simulink model "HPPC"  (R2026a)
settings: Solver=FixedStepDiscrete  StopTime=inf  FixedStep=Ts
model workspace (MATLAB code in the model file):
  | % Defaults for standalone use and code generation, from HPP_parameters.
  | % In HPP.slx the Model block passes p.ctrl.hppc.par as the argument "par".
  | pDefault = HPP_parameters();
  | Ts  = pDefault.ctrl.hppc.Ts;    % [s] fixed sample time
  | par = pDefault.ctrl.hppc.par;   % tunable parameters (model argument)
  | clear pDefault
libraries: simulink x5, slpidlib x2, sl_discontinuities x1
Description:
  | HPP controller (stage 5, Energinet DK1): P set-point with ramp rate constraint, frequency response (LFSM-O, LFSM-U, optional FSM with reserve; Frqflag) added after the ramp limit, export limit; closed-loop P at the POC (PI on P_target - P_poc, target fed forward, Pflag); SOC-aware BESS limits; dispatch: wind and PV at available power, the BESS balances, wind and PV curtailed when the BESS cannot absorb more. Q control (Q_ref), voltage control (Vref, slope Vslope) or power factor control (PF) at the POC with PI (Qflag, RefFlag 0 / 1 / 2), Q order split over the plants by rating. Both PIs frozen in a voltage dip. Per unit on p.ctrl.hppc.Pbase. Parameters: model argument par (= p.ctrl.hppc.par, from p.hppc).
settings Model: ParameterArgumentNames=par  Creator=kjaer  LastModifiedBy=kjaer

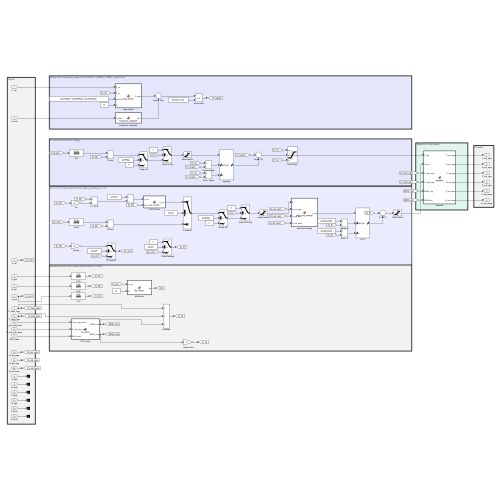
[thumbnail: Simulink's stored preview of the top-level diagram]
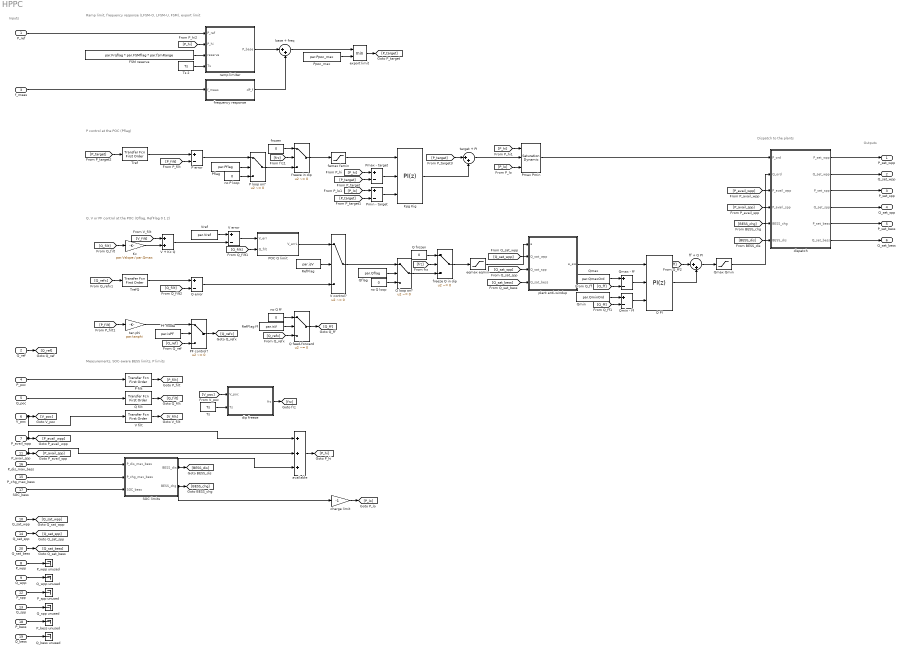
== system HPPC ==
  note: Inputs
  note: Ramp limit, frequency response (LFSM-O, LFSM-U, FSM), export limit
  note: P control at the POC (Pflag)
  note: Q, V or PF control at the POC (Qflag, RefFlag 0 1 2)
  note: Measurements, SOC-aware BESS limits, P limits
  note: Dispatch to the plants
  note: Outputs
  P_ref : Inport  OutDataTypeStr=double  PortDimensions=1  SampleTime=Ts
  Q_ref : Inport  Port=2  OutDataTypeStr=double  PortDimensions=1  SampleTime=Ts
  f_meas : Inport  Port=3  OutDataTypeStr=double  PortDimensions=1  SampleTime=Ts
  P_poc : Inport  Port=4  OutDataTypeStr=double  PortDimensions=1  SampleTime=Ts
  Q_poc : Inport  Port=5  OutDataTypeStr=double  PortDimensions=1  SampleTime=Ts
  V_poc : Inport  Port=6  OutDataTypeStr=double  PortDimensions=1  SampleTime=Ts
  P_avail_wpp : Inport  Port=7  OutDataTypeStr=double  PortDimensions=1  SampleTime=Ts
  P_wpp : Inport  Port=8  OutDataTypeStr=double  PortDimensions=1  SampleTime=Ts
  Q_wpp : Inport  Port=9  OutDataTypeStr=double  PortDimensions=1  SampleTime=Ts
  Q_sat_wpp : Inport  Port=10  OutDataTypeStr=double  PortDimensions=1  SampleTime=Ts
  P_avail_spp : Inport  Port=11  OutDataTypeStr=double  PortDimensions=1  SampleTime=Ts
  P_spp : Inport  Port=12  OutDataTypeStr=double  PortDimensions=1  SampleTime=Ts
  Q_spp : Inport  Port=13  OutDataTypeStr=double  PortDimensions=1  SampleTime=Ts
  Q_sat_spp : Inport  Port=14  OutDataTypeStr=double  PortDimensions=1  SampleTime=Ts
  P_chg_max_bess : Inport  Port=15  OutDataTypeStr=double  PortDimensions=1  SampleTime=Ts
  P_dis_max_bess : Inport  Port=16  OutDataTypeStr=double  PortDimensions=1  SampleTime=Ts
  SOC_bess : Inport  Port=17  OutDataTypeStr=double  PortDimensions=1  SampleTime=Ts
  P_bess : Inport  Port=18  OutDataTypeStr=double  PortDimensions=1  SampleTime=Ts
  Q_bess : Inport  Port=19  OutDataTypeStr=double  PortDimensions=1  SampleTime=Ts
  Q_sat_bess : Inport  Port=20  OutDataTypeStr=double  PortDimensions=1  SampleTime=Ts
  FSM reserve : Constant  Value=par.Frqflag * par.FSMflag * par.fsmRange
  Kc : Gain  Gain=par.Vslope / par.Qmax
  Kpg Kig : slpidlib/PID Controller  Controller=PI  Form=Parallel  TimeDomain=Discrete-time  UseExternalTs=off  SampleTime=-1  IntegratorMethod=Forward Euler  FilterMethod=Forward Euler  ControllerParametersSource=internal  P=par.Kpg  I=par.Kig  UseKiTs=off  D=0  UseExternalDerivativeSource=off  N=100  UseFilter=on  TunerSelectOption=Transfer Function Based (PID Tuner App)  InitialConditionSource=internal  InitialConditionForIntegrator=0  InitialConditionForFilter=0  DifferentiatorICPrevScaledInput=0  ExternalReset=none  TrackingMode=off  Kt=1  LimitOutput=on  SatLimitsSource=external  UpperSaturationLimit=inf  LowerSaturationLimit=-inf  LinearizeAsGain=off  AntiWindupMode=clamping  Kb=1  LimitIntegrator=off  UpperIntegratorSaturationLimit=inf  LowerIntegratorSaturationLimit=-inf  POutMin=[]  POutMax=[]  IOutMin=[]  IOutMax=[]  DOutMin=[]  DOutMax=[]  NOutMin=[]  NOutMax=[]  SumOutMin=[]  SumOutMax=[]  SaturationOutMin=[]  SaturationOutMax=[]  PParamMin=[]  PParamMax=[]  IParamMin=[]  IParamMax=[]  DParamMin=[]  DParamMax=[]  NParamMin=[]  NParamMax=[]  KbParamMin=[]  KbParamMax=[]  KtParamMin=[]  KtParamMax=[]  KbOutMin=[]  KbOutMax=[]  KtOutMin=[]  KtOutMax=[]  IntegratorOutMin=[]  IntegratorOutMax=[]  FilterOutMin=[]  FilterOutMax=[]  SumI1OutMin=[]  SumI1OutMax=[]  SumI2OutMin=[]  SumI2OutMax=[]  SumI3OutMin=[]  SumI3OutMax=[]  SumI4OutMin=[]  SumI4OutMax=[]  SumDOutMin=[]  SumDOutMax=[]  DifferentiatorOutMin=[]  DifferentiatorOutMax=[]  FilterDiffOutCoefMin=[]  FilterDiffOutCoefMax=[]  ReciprocalOutMin=[]  ReciprocalOutMax=[]  SumDenOutMin=[]  SumDenOutMax=[]  SumNumOutMin=[]  SumNumOutMax=[]  DivideOutMin=[]  DivideOutMax=[]  UdiffTsProdOutMin=[]  UdiffTsProdOutMax=[]  NTsProdOutMin=[]  NTsProdOutMax=[]  UintegralTsProdOutMin=[]  UintegralTsProdOutMax=[]  UngainTsProdOutMin=[]  UngainTsProdOutMax=[]  ClampingZeroOutDataTypeStr=Inherit: Inherit via back propagation  ClampingZeroOutMin=[]  ClampingZeroOutMax=[]  FilterDenConstantOutDataTypeStr=Inherit: Inherit via back propagation  FilterDenConstantOutMin=[]  FilterDenConstantOutMax=[]  PCopyOutDataTypeStr=Inherit: Inherit via back propagation  PCopyOutMin=[]  PCopyOutMax=[]  NCopyOutDataTypeStr=Inherit: Inherit via back propagation  NCopyOutMin=[]  NCopyOutMax=[]  IntegratorContinuousStateAttributes=''  IntegratorStateMustResolveToSignalObject=off  IntegratorRTWStateStorageClass=Auto  FilterContinuousStateAttributes=''  FilterStateMustResolveToSignalObject=off  FilterRTWStateStorageClass=Auto  ParallelPVariant=InternalParameters  IdealPVariant=Disabled  IVariant=InternalParameters  DVariant=Disabled  IntegratorVariant=Discrete  SatVariant=External  AWVariant=DiscClampingParallel  PCopyVariant=Disabled  TRVariant=Disabled  FdbkBlocksVariant=Forward  IdealPFdbkVariant=Disabled  SatFdbkVariant=Disabled  DerivativeFilterVariant=Disabled  NVariant=Disabled  NCopyVariant=Disabled_SignalSpec  FilterICVariant=Disabled  IntegratorICVariant=InternalICs  ExternalResetVariant=Disabled  TRSumVariant=Passthrough  SumFdbkVariant=Disabled  SumVariant=Sum_PI  TsampFilterVariant=InternalTs  TsampNgainVariant=Passthrough  TsampIntegralVariant=Disabled_SignalSpec  ExternalSaturationOutDataTypeStr=Inherit: Same as second input  DerivativeSourceVariant=Disabled  PreIntVariant=InternalPreInt
      settings: LibrarySourceBlock=simulink/Discrete/Discrete PID Controller
  P error : Sum  Inputs=+-
  P filt : simulink/Discrete/Transfer Fcn First Order  PoleZ=1 - Ts/par.Tp  ICPrevOutput=0  DoSatur=off
  P loop on? : Switch  Criteria=u2 ~= 0  SaturateOnIntegerOverflow=off  InputSameDT=off
  PF control? : Switch  Criteria=u2 ~= 0  SaturateOnIntegerOverflow=off  InputSameDT=off
  PF mode : Constant  Value=par.isPF
  POC Q limit : MATLAB Function  TreatAsAtomicUnit=on
  P_bess unused : Terminator
  P_spp unused : Terminator
  P_wpp unused : Terminator
  Pflag : Constant  Value=par.Pflag
  Pmax - target : Sum  Inputs=+-
  Pmax Pmin : sl_discontinuities/Saturation Dynamic  OutMin=[]  OutMax=[]  OutDataTypeStr=Inherit: Same as second input  OutDataType=fixdt(1, 16)  OutScaling=2^-10  DoSatur=off
      settings: LibrarySourceBlock=|
      | simulink/Discontinuities/Saturation
      | Dynamic
  Pmin - target : Sum  Inputs=+-
  Ppoc_max : Constant  Value=par.Ppoc_max
  Q PI : slpidlib/PID Controller  Controller=PI  Form=Parallel  TimeDomain=Discrete-time  UseExternalTs=off  SampleTime=-1  IntegratorMethod=Forward Euler  FilterMethod=Forward Euler  ControllerParametersSource=internal  P=par.KpQ  I=par.KiQ  UseKiTs=off  D=0  UseExternalDerivativeSource=off  N=100  UseFilter=on  TunerSelectOption=Transfer Function Based (PID Tuner App)  InitialConditionSource=internal  InitialConditionForIntegrator=0  InitialConditionForFilter=0  DifferentiatorICPrevScaledInput=0  ExternalReset=none  TrackingMode=off  Kt=1  LimitOutput=on  SatLimitsSource=external  UpperSaturationLimit=inf  LowerSaturationLimit=-inf  LinearizeAsGain=off  AntiWindupMode=clamping  Kb=1  LimitIntegrator=off  UpperIntegratorSaturationLimit=inf  LowerIntegratorSaturationLimit=-inf  POutMin=[]  POutMax=[]  IOutMin=[]  IOutMax=[]  DOutMin=[]  DOutMax=[]  NOutMin=[]  NOutMax=[]  SumOutMin=[]  SumOutMax=[]  SaturationOutMin=[]  SaturationOutMax=[]  PParamMin=[]  PParamMax=[]  IParamMin=[]  IParamMax=[]  DParamMin=[]  DParamMax=[]  NParamMin=[]  NParamMax=[]  KbParamMin=[]  KbParamMax=[]  KtParamMin=[]  KtParamMax=[]  KbOutMin=[]  KbOutMax=[]  KtOutMin=[]  KtOutMax=[]  IntegratorOutMin=[]  IntegratorOutMax=[]  FilterOutMin=[]  FilterOutMax=[]  SumI1OutMin=[]  SumI1OutMax=[]  SumI2OutMin=[]  SumI2OutMax=[]  SumI3OutMin=[]  SumI3OutMax=[]  SumI4OutMin=[]  SumI4OutMax=[]  SumDOutMin=[]  SumDOutMax=[]  DifferentiatorOutMin=[]  DifferentiatorOutMax=[]  FilterDiffOutCoefMin=[]  FilterDiffOutCoefMax=[]  ReciprocalOutMin=[]  ReciprocalOutMax=[]  SumDenOutMin=[]  SumDenOutMax=[]  SumNumOutMin=[]  SumNumOutMax=[]  DivideOutMin=[]  DivideOutMax=[]  UdiffTsProdOutMin=[]  UdiffTsProdOutMax=[]  NTsProdOutMin=[]  NTsProdOutMax=[]  UintegralTsProdOutMin=[]  UintegralTsProdOutMax=[]  UngainTsProdOutMin=[]  UngainTsProdOutMax=[]  ClampingZeroOutDataTypeStr=Inherit: Inherit via back propagation  ClampingZeroOutMin=[]  ClampingZeroOutMax=[]  FilterDenConstantOutDataTypeStr=Inherit: Inherit via back propagation  FilterDenConstantOutMin=[]  FilterDenConstantOutMax=[]  PCopyOutDataTypeStr=Inherit: Inherit via back propagation  PCopyOutMin=[]  PCopyOutMax=[]  NCopyOutDataTypeStr=Inherit: Inherit via back propagation  NCopyOutMin=[]  NCopyOutMax=[]  IntegratorContinuousStateAttributes=''  IntegratorStateMustResolveToSignalObject=off  IntegratorRTWStateStorageClass=Auto  FilterContinuousStateAttributes=''  FilterStateMustResolveToSignalObject=off  FilterRTWStateStorageClass=Auto  ParallelPVariant=InternalParameters  IdealPVariant=Disabled  IVariant=InternalParameters  DVariant=Disabled  IntegratorVariant=Discrete  SatVariant=External  AWVariant=DiscClampingParallel  PCopyVariant=Disabled  TRVariant=Disabled  FdbkBlocksVariant=Forward  IdealPFdbkVariant=Disabled  SatFdbkVariant=Disabled  DerivativeFilterVariant=Disabled  NVariant=Disabled  NCopyVariant=Disabled_SignalSpec  FilterICVariant=Disabled  IntegratorICVariant=InternalICs  ExternalResetVariant=Disabled  TRSumVariant=Passthrough  SumFdbkVariant=Disabled  SumVariant=Sum_PI  TsampFilterVariant=InternalTs  TsampNgainVariant=Passthrough  TsampIntegralVariant=Disabled_SignalSpec  ExternalSaturationOutDataTypeStr=Inherit: Same as second input  DerivativeSourceVariant=Disabled  PreIntVariant=InternalPreInt
      settings: LibrarySourceBlock=simulink/Discrete/Discrete PID Controller
  Q error : Sum  Inputs=+-
  Q feed-forward : Switch  Criteria=u2 ~= 0  SaturateOnIntegerOverflow=off  InputSameDT=off
  Q filt : simulink/Discrete/Transfer Fcn First Order  PoleZ=1 - Ts/par.Tq  ICPrevOutput=0  DoSatur=off
  Q frozen : Constant  Value=0
  Q loop on? : Switch  Criteria=u2 ~= 0  SaturateOnIntegerOverflow=off  InputSameDT=off
  Q_bess unused : Terminator
  Q_spp unused : Terminator
  Q_wpp unused : Terminator
  Qflag : Constant  Value=par.Qflag
  Qmax : Constant  Value=par.QmaxOrd
  Qmax - ff : Sum  Inputs=+-
  Qmax Qmin : Saturate  UpperLimit=par.QmaxOrd  LowerLimit=par.QminOrd
  Qmin : Constant  Value=par.QminOrd
  Qmin - ff : Sum  Inputs=+-
  RefFlag : Constant  Value=par.isV
  RefFlag ff : Constant  Value=par.isV
  SOC limits : MATLAB Function  TreatAsAtomicUnit=on
  Tref : simulink/Discrete/Transfer Fcn First Order  PoleZ=1 - Ts/par.Tref  ICPrevOutput=0  DoSatur=off
  TrefQ : simulink/Discrete/Transfer Fcn First Order  PoleZ=1 - Ts/par.TrefQ  ICPrevOutput=0  DoSatur=off
  Ts : Constant  Value=Ts
  Ts 2 : Constant  Value=Ts
  V + Kc Q : Sum
  V control? : Switch  Criteria=u2 ~= 0  SaturateOnIntegerOverflow=off  InputSameDT=off
  V error : Sum  Inputs=+-
  V filt : simulink/Discrete/Transfer Fcn First Order  PoleZ=1 - Ts/par.Tq  ICPrevOutput=1  DoSatur=off
  Vref : Constant  Value=par.Vref
  available : Sum  Inputs=+++
  base + freq : Sum  Inputs=|++
  charge limit : Gain  Gain=-1
  dip freeze : MATLAB Function  TreatAsAtomicUnit=on
  dispatch : MATLAB Function  TreatAsAtomicUnit=on
  eqmax eqmin : Saturate  UpperLimit=par.eqmax  LowerLimit=par.eqmin
  export limit : MinMax  Inputs=2
  femax femin : Saturate  UpperLimit=par.femax  LowerLimit=par.femin
  ff + Q PI : Sum  Inputs=|++
  freeze Q in dip : Switch  Criteria=u2 ~= 0  SaturateOnIntegerOverflow=off  InputSameDT=off
  freeze in dip : Switch  Criteria=u2 ~= 0  SaturateOnIntegerOverflow=off  InputSameDT=off
  frequency response : MATLAB Function  TreatAsAtomicUnit=on
  frozen : Constant  Value=0
  no P loop : Constant  Value=0
  no Q ff : Constant  Value=0
  no Q loop : Constant  Value=0
  plant anti-windup : MATLAB Function  TreatAsAtomicUnit=on
  ramp limiter : MATLAB Function  TreatAsAtomicUnit=on
  tan phi : Gain  Gain=par.tanphi
  target + PI : Sum  Inputs=|++
  P_set_wpp : Outport  OutDataTypeStr=double
  Q_set_wpp : Outport  Port=2  OutDataTypeStr=double
  P_set_spp : Outport  Port=3  OutDataTypeStr=double
  Q_set_spp : Outport  Port=4  OutDataTypeStr=double
  P_set_bess : Outport  Port=5  OutDataTypeStr=double
  Q_set_bess : Outport  Port=6  OutDataTypeStr=double
  wires:
  P filt/1 -> [P_filt]
  [P_filt] -> P error/2
  [P_filt] -> tan phi/1
  PF control?/1 -> [Q_refx]
  [Q_refx] -> Q feed-forward/3
  [Q_refx] -> TrefQ/1
  P_avail_spp/1 -> [P_avail_spp], available/2
  [P_avail_spp] -> dispatch/4(P_avail_spp)
  P_avail_wpp/1 -> [P_avail_wpp], available/1
  [P_avail_wpp] -> dispatch/3(P_avail_wpp)
  Q feed-forward/1 -> [Q_ff]
  [Q_ff] -> Qmax - ff/2
  [Q_ff] -> Qmin - ff/2
  [Q_ff] -> ff + Q PI/1
  Q filt/1 -> [Q_filt]
  [Q_filt] -> Kc/1
  [Q_filt] -> POC Q limit/2(Q_filt)
  [Q_filt] -> Q error/2
  Q_ref/1 -> [Q_ref]
  [Q_ref] -> PF control?/3
  Q_sat_bess/1 -> [Q_sat_bess]
  [Q_sat_bess] -> plant anti-windup/4(Q_sat_bess)
  Q_sat_spp/1 -> [Q_sat_spp]
  [Q_sat_spp] -> plant anti-windup/3(Q_sat_spp)
  Q_sat_wpp/1 -> [Q_sat_wpp]
  [Q_sat_wpp] -> plant anti-windup/2(Q_sat_wpp)
  SOC limits/1(BESS_dis) -> [BESS_dis], available/3
  [BESS_dis] -> dispatch/6(BESS_dis)
  SOC limits/2(BESS_chg) -> [BESS_chg], charge limit/1
  [BESS_chg] -> dispatch/5(BESS_chg)
  V filt/1 -> [V_filt]
  [V_filt] -> V + Kc Q/1
  V_poc/1 -> [V_poc], V filt/1
  [V_poc] -> dip freeze/1(V_poc)
  available/1 -> [P_hi]
  [P_hi] -> Pmax - target/1
  [P_hi] -> Pmax Pmin/1
  [P_hi] -> ramp limiter/2(P_hi)
  charge limit/1 -> [P_lo]
  [P_lo] -> Pmax Pmin/3
  [P_lo] -> Pmin - target/1
  dip freeze/1(frz) -> [frz]
  [frz] -> freeze Q in dip/2
  [frz] -> freeze in dip/2
  export limit/1 -> [P_target]
  [P_target] -> Pmax - target/2
  [P_target] -> Pmin - target/2
  [P_target] -> Tref/1
  [P_target] -> target + PI/1
  FSM reserve/1 -> ramp limiter/3(reserve)
  Kc/1 -> V + Kc Q/2
  Kpg Kig/1 -> target + PI/2
  P error/1 -> P loop on?/1
  P loop on?/1 -> freeze in dip/3
  PF mode/1 -> PF control?/2
  POC Q limit/1(V_errL) -> V control?/1
  P_bess/1 -> P_bess unused/1
  P_chg_max_bess/1 -> SOC limits/2(P_chg_max_bess)
  P_dis_max_bess/1 -> SOC limits/1(P_dis_max_bess)
  P_poc/1 -> P filt/1
  P_ref/1 -> ramp limiter/1(P_ref)
  P_spp/1 -> P_spp unused/1
  P_wpp/1 -> P_wpp unused/1
  Pflag/1 -> P loop on?/2
  Pmax - target/1 -> Kpg Kig/2
  Pmax Pmin/1 -> dispatch/1(P_ord)
  Pmin - target/1 -> Kpg Kig/3
  Ppoc_max/1 -> export limit/2
  Q PI/1 -> ff + Q PI/2
  Q error/1 -> V control?/3
  Q frozen/1 -> freeze Q in dip/1
  Q loop on?/1 -> freeze Q in dip/3
  Q_bess/1 -> Q_bess unused/1
  Q_poc/1 -> Q filt/1
  Q_spp/1 -> Q_spp unused/1
  Q_wpp/1 -> Q_wpp unused/1
  Qflag/1 -> Q loop on?/2
  Qmax - ff/1 -> Q PI/2
  Qmax Qmin/1 -> dispatch/2(Q_ord)
  Qmax/1 -> Qmax - ff/1
  Qmin - ff/1 -> Q PI/3
  Qmin/1 -> Qmin - ff/1
  RefFlag ff/1 -> Q feed-forward/2
  RefFlag/1 -> V control?/2
  SOC_bess/1 -> SOC limits/3(SOC_bess)
  Tref/1 -> P error/1
  TrefQ/1 -> Q error/1
  Ts 2/1 -> ramp limiter/4(Ts)
  Ts/1 -> dip freeze/2(Ts)
  V + Kc Q/1 -> V error/2
  V control?/1 -> Q loop on?/1
  V error/1 -> POC Q limit/1(V_err)
  Vref/1 -> V error/1
  base + freq/1 -> export limit/1
  dispatch/1(P_set_wpp) -> P_set_wpp/1
  dispatch/2(Q_set_wpp) -> Q_set_wpp/1
  dispatch/3(P_set_spp) -> P_set_spp/1
  dispatch/4(Q_set_spp) -> Q_set_spp/1
  dispatch/5(P_set_bess) -> P_set_bess/1
  dispatch/6(Q_set_bess) -> Q_set_bess/1
  eqmax eqmin/1 -> plant anti-windup/1(e)
  f_meas/1 -> frequency response/1(f_meas)
  femax femin/1 -> Kpg Kig/1
  ff + Q PI/1 -> Qmax Qmin/1
  freeze Q in dip/1 -> eqmax eqmin/1
  freeze in dip/1 -> femax femin/1
  frequency response/1(dP_f) -> base + freq/2
  frozen/1 -> freeze in dip/1
  no P loop/1 -> P loop on?/3
  no Q ff/1 -> Q feed-forward/1
  no Q loop/1 -> Q loop on?/3
  plant anti-windup/1(e_aw) -> Q PI/1
  ramp limiter/1(P_base) -> base + freq/1
  tan phi/1 -> PF control?/1
  target + PI/1 -> Pmax Pmin/2

== matlab function HPPC/dip freeze ==
  data: V_poc input; frz output; Ts input; par parameter
function frz  = dip_freeze(V_poc, Ts, par)
%#codegen
% Freeze the P loop while the POC voltage is below Vfrz (voltage dip)
% and for Thld after it, while the assets recover their active power.
persistent n
if isempty(n), n = 0; end
if V_poc < par.Vfrz
    n = round(par.Thld / Ts);
elseif n > 0
    n = n - 1;
end
frz = double(V_poc < par.Vfrz || n > 0);
end

== matlab function HPPC/SOC limits ==
  data: P_dis_max_bess input; BESS_dis output; P_chg_max_bess input; SOC_bess input; BESS_chg output; par parameter
function [BESS_dis, BESS_chg] = soc_limits(P_dis_max_bess, P_chg_max_bess, SOC_bess, par)
%#codegen
% SOC-aware BESS limits: discharge (charge) derated linearly to zero
% over SOCband above SOCmin (below SOCmax), so the BESS approaches its
% SOC limits smoothly instead of stopping at them.
kd = min(max((SOC_bess - par.SOCmin) / par.SOCband, 0), 1);
kc = min(max((par.SOCmax - SOC_bess) / par.SOCband, 0), 1);
BESS_dis = P_dis_max_bess * kd;
BESS_chg = P_chg_max_bess * kc;
end

== matlab function HPPC/ramp limiter ==
  data: P_ref input; P_base output; P_hi input; reserve input; Ts input; par parameter
function P_base  = ramp_limiter(P_ref, P_hi, reserve, Ts, par)
%#codegen
% Base P order: the TSO set-point, limited to what the plant can deliver
% while keeping the FSM reserve, with the ramp rate constraint (rampUp,
% rampDn in pu of Pn per minute). Starts at the set-point.
persistent y
if isempty(y), y = P_ref; end
u = min(P_ref, max(P_hi - reserve, 0));
if par.rampFlag
    y = y + min(max(u - y, -par.rampDn / 60 * Ts), par.rampUp / 60 * Ts);
else
    y = u;
end
P_base = y;
end

== matlab function HPPC/frequency response ==
  data: f_meas input; dP_f output; par parameter
function dP_f  = frequency_response(f_meas, par)
%#codegen
% Active power frequency response, pu of Pn (= POC base) per pu of f:
% LFSM-O above fO (droop sO) and LFSM-U below fU (droop sU), always on;
% FSM (FSMflag, FCR delivery): droop sFSM with deadband fsmDb, limited
% to +-fsmRange. Frqflag 0 switches all of it off (decentral cases).
df = f_meas - par.Freq_ref;
dP = 0;
if par.FSMflag
    e = sign(df) * max(abs(df) - par.fsmDb, 0);
    dP = min(max(-e / par.sFSM, -par.fsmRange), par.fsmRange);
end
dP = dP - max(f_meas - par.fO, 0) / par.sO + max(par.fU - f_meas, 0) / par.sU;
dP_f = par.Frqflag * dP;
end

== matlab function HPPC/POC Q limit ==
  data: V_err input; V_errL output; Q_filt input; par parameter
function V_errL  = poc_q_limit(V_err, Q_filt, par)
%#codegen
% Q limit at the POC in voltage control: where the slope asks for more
% than Qmax (less than Qmin), the voltage error is capped by the Q margin,
% scaled by the loop gain (V error per Q), so the loop settles at the
% limit. Needed with local voltage control in the plants, where the HPPC
% order is only the offset of their droop lines.
k = par.Vslope / par.Qmax + par.dVdQ;
V_errL = min(max(V_err, (par.Qmin - Q_filt) * k), (par.Qmax - Q_filt) * k);
end

== matlab function HPPC/plant anti-windup ==
  data: e input; e_aw output; Q_sat_wpp input; Q_sat_spp input; Q_sat_bess input; par parameter
function e_aw  = plant_anti_windup(e, Q_sat_wpp, Q_sat_spp, Q_sat_bess, par)
%#codegen
% Anti-windup over the plant limits (conditional integration): the HPPC
% order is split over all plants, so when every plant reports its Q order
% at the upper (lower) limit, more (less) order cannot change Q: hold the
% Q loop (error 0) in that direction. Plants' own limits are inside the
% plant controllers; this is how the HPPC learns about them.
up = Q_sat_wpp > 0.5 && Q_sat_spp > 0.5 && Q_sat_bess > 0.5;
dn = Q_sat_wpp < -0.5 && Q_sat_spp < -0.5 && Q_sat_bess < -0.5;
e_aw = e;
if par.QawFlag && ((e > 0 && up) || (e < 0 && dn))
    e_aw = 0;
end
end

== matlab function HPPC/dispatch ==
  data: P_ord input; P_set_wpp output; Q_ord input; P_avail_wpp input; P_avail_spp input; BESS_chg input; BESS_dis input; Q_set_wpp output; P_set_spp output; Q_set_spp output; P_set_bess output; Q_set_bess output; par parameter
function [P_set_wpp, Q_set_wpp, P_set_spp, Q_set_spp, P_set_bess, Q_set_bess] = dispatch(P_ord, Q_ord, P_avail_wpp, P_avail_spp, BESS_chg, BESS_dis, par)
%#codegen
% P: wind and PV at available power, the BESS balances the rest within
% its SOC-aware charge / discharge limits; wind and PV are curtailed (in
% proportion to their availability) only when the BESS cannot absorb the
% surplus (also when it is nearly full).
% Q: the HPPC's Q order split over the plants by rating.
P_ren = P_avail_wpp + P_avail_spp;
P_set_bess = min(max(P_ord - P_ren, -BESS_chg), BESS_dis);
P_r = min(max(P_ord - P_set_bess, 0), P_ren);
if P_ren > 1e-6
    w = P_avail_wpp / P_ren;
else
    w = par.qshare(1) / (par.qshare(1) + par.qshare(2));
end
P_set_wpp = P_r * w;
P_set_spp = P_r * (1 - w);
Q_set_wpp  = Q_ord * par.qshare(1);
Q_set_spp  = Q_ord * par.qshare(2);
Q_set_bess = Q_ord * par.qshare(3);
end
